simulink model "BMS_OC_Integration_Reset_Test"  (R2025b)
settings: Solver=FixedStepDiscrete  StartTime=0.0  StopTime=1  FixedStep=Ts  RelTol=1e-3
InitFcn:
  | init_BMS
undefined symbols (not defined in the file): Ts
libraries: BMS_Library x1
settings Model: Creator=Khadija  LastModifiedBy=Khadija

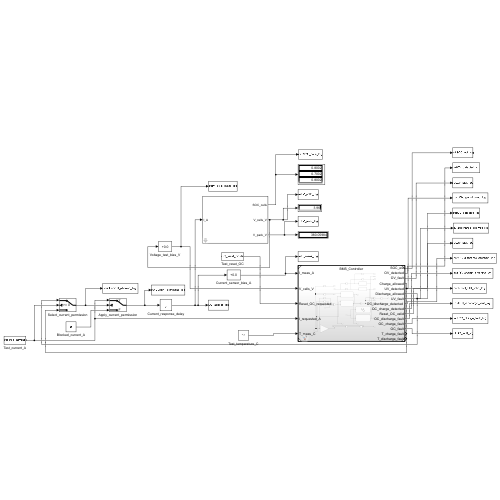
[thumbnail: Simulink's stored preview of the top-level diagram]
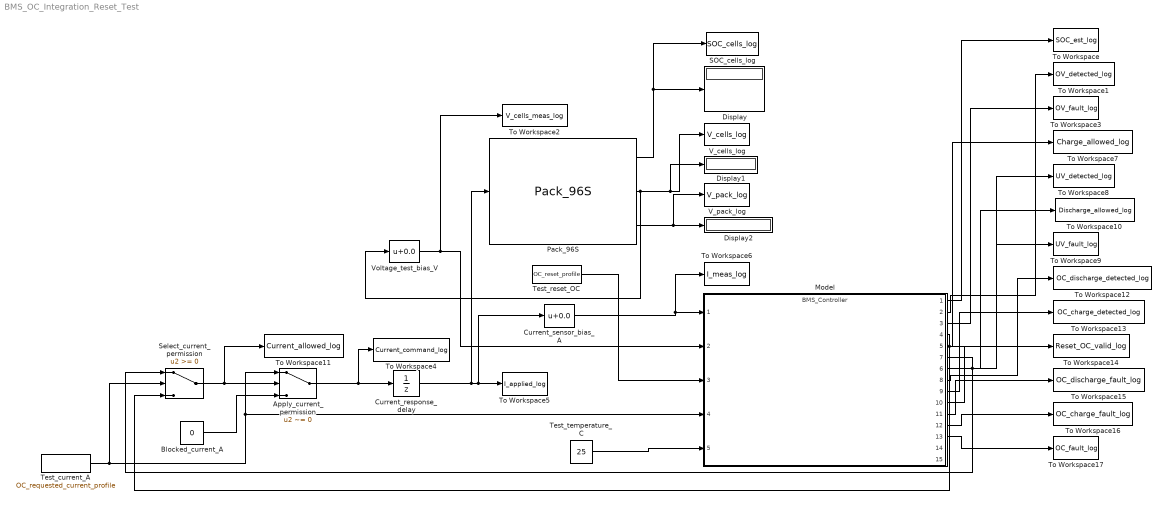
== system BMS_OC_Integration_Reset_Test ==
  Apply_current_permission : Switch  Criteria=u2 ~= 0  SaturateOnIntegerOverflow=off  InputSameDT=off
  Blocked_current_A : Constant  Value=0  SampleTime=Ts
  Current_response_delay : UnitDelay  SampleTime=Ts  HasFrameUpgradeWarning=on
  Current_sensor_bias_A : Bias  Bias=0.0  SaturateOnIntegerOverflow=off
  Display : Display
  Display1 : Display
  Display2 : Display
  Model : ModelReference  ModelNameDialog=BMS_Controller  SimulationMode=Normal  ModelReferenceVersion=1.40
      settings: PortSchema="{\"entries\":[{\"content\":{\"sides\":[{\"content\":{\"connectorIds\":[\"In1\",\"In2\",\"In3\",\"In4\",\"In5\"]},\"type\":\"ConnectorPlacement.EquallySpacedRectSide\",\"uuid\":\"1e26f145-0f3d-496d-921d-7ad329268fcb\"},{\"content\":{\"connectorIds\":[\"Out1\",\"Out2\",\"Out3\",\"Out4\",\"Out5\",\"Out7\",\"Out6\",\"Out8\",\"Out9\",\"Out10\",\"Out11\",\"Out12\",\"Out13\",\"Out14\",\"Out15\"],\"side\":\"RIGHT\"},\"type\":\"ConnectorPlacement.EquallySpacedRectSide\",\"uuid\":\"f623cd1b-04b5-4ae4-86fc-b9e653a015f6\"},{\"content\":{\"side\":\"TOP\"},\"type\":\"ConnectorPlacement.EquallySpacedRectSide\",\"uuid\":\"e3a00977-f6c2-4554-bcd2-84dd8f01a2c6\"}]},\"type\":\"ConnectorPlacement.EquallySpacedConnector\",\"uuid\":\"60ffb283-705f-43a9-b3aa-b4ebe7e6c32d\"}],\"packageUris\":[\"http://schema.mathworks.com/mf0/Connector/R2020b\"],\"version\":\"1.0\"}"
  Pack_96S : BMS_Library/Pack_96S  SOC_init_pack=SOC0_pack
  SOC_cells_log : ToWorkspace  VariableName=SOC_cells_log  SaveFormat=Timeseries  SampleTime=-1
  Select_current_permission : Switch  SaturateOnIntegerOverflow=off  InputSameDT=off
  Test_current_A : FromWorkspace  VariableName=OC_requested_current_profile  OutDataTypeStr=double  SampleTime=Ts  Interpolate=off  OutputAfterFinalValue=Holding final value
  Test_reset_OC : FromWorkspace  VariableName=OC_reset_profile  OutDataTypeStr=boolean  SampleTime=Ts  Interpolate=off  OutputAfterFinalValue=Holding final value
  Test_temperature_C : Constant  Value=25  OutDataTypeStr=double  SampleTime=Ts
  To Workspace : ToWorkspace  VariableName=SOC_est_log  SaveFormat=Timeseries  SampleTime=-1
  To Workspace1 : ToWorkspace  VariableName=OV_detected_log  SaveFormat=Timeseries  SampleTime=-1
  To Workspace10 : ToWorkspace  VariableName=Discharge_allowed_log  SaveFormat=Timeseries  SampleTime=-1
  To Workspace11 : ToWorkspace  VariableName=Current_allowed_log  SaveFormat=Timeseries  SampleTime=-1
  To Workspace12 : ToWorkspace  VariableName=OC_discharge_detected_log  SaveFormat=Timeseries  SampleTime=-1
  To Workspace13 : ToWorkspace  VariableName=OC_charge_detected_log  SaveFormat=Timeseries  SampleTime=-1
  To Workspace14 : ToWorkspace  VariableName=Reset_OC_valid_log  SaveFormat=Timeseries  SampleTime=-1
  To Workspace15 : ToWorkspace  VariableName=OC_discharge_fault_log  SaveFormat=Timeseries  SampleTime=-1
  To Workspace16 : ToWorkspace  VariableName=OC_charge_fault_log  SaveFormat=Timeseries  SampleTime=-1
  To Workspace17 : ToWorkspace  VariableName=OC_fault_log  SaveFormat=Timeseries  SampleTime=-1
  To Workspace2 : ToWorkspace  VariableName=V_cells_meas_log  SaveFormat=Timeseries  SampleTime=-1
  To Workspace3 : ToWorkspace  VariableName=OV_fault_log  SaveFormat=Timeseries  SampleTime=-1
  To Workspace4 : ToWorkspace  VariableName=Current_command_log  SaveFormat=Timeseries  SampleTime=-1
  To Workspace5 : ToWorkspace  VariableName=I_applied_log  SaveFormat=Timeseries  SampleTime=-1
  To Workspace6 : ToWorkspace  VariableName=I_meas_log  SaveFormat=Timeseries  SampleTime=-1
  To Workspace7 : ToWorkspace  VariableName=Charge_allowed_log  SaveFormat=Timeseries  SampleTime=-1
  To Workspace8 : ToWorkspace  VariableName=UV_detected_log  SaveFormat=Timeseries  SampleTime=-1
  To Workspace9 : ToWorkspace  VariableName=UV_fault_log  SaveFormat=Timeseries  SampleTime=-1
  V_cells_log : ToWorkspace  VariableName=V_cells_log  SaveFormat=Timeseries  SampleTime=-1
  V_pack_log : ToWorkspace  VariableName=V_pack_log  SaveFormat=Timeseries  SampleTime=-1
  Voltage_test_bias_V : Bias  Bias=0.0  SaturateOnIntegerOverflow=off
  wires:
  Select_current_permission/1 -> To Workspace11/1, Apply_current_permission/2
  Test_current_A/1 -> Apply_current_permission/1, Model/4, Select_current_permission/2
  Current_response_delay/1 -> To Workspace5/1, Current_sensor_bias_A/1, Pack_96S/1
  Apply_current_permission/1 -> To Workspace4/1, Current_response_delay/1
  Blocked_current_A/1 -> Apply_current_permission/3
  Voltage_test_bias_V/1 -> Model/2, To Workspace2/1
  Model/13 -> To Workspace17/1
  Model/9 -> To Workspace13/1
  Model/5 -> To Workspace8/1
  Pack_96S/2 -> Display1/1, V_cells_log/1, Voltage_test_bias_V/1
  Model/12 -> To Workspace16/1
  Model/8 -> To Workspace12/1
  Model/4 -> Select_current_permission/3, To Workspace7/1
  Pack_96S/1 -> SOC_cells_log/1, Display/1
  Model/10 -> To Workspace14/1
  Model/6 -> To Workspace9/1
  Pack_96S/3 -> V_pack_log/1, Display2/1
  Test_reset_OC/1 -> Model/3
  Model/1 -> To Workspace/1
  Current_sensor_bias_A/1 -> To Workspace6/1, Model/1
  Model/2 -> To Workspace1/1
  Model/3 -> To Workspace3/1
  Model/11 -> To Workspace15/1
  Model/7 -> Select_current_permission/1, To Workspace10/1
  Test_temperature_C/1 -> Model/5
